simulink model "exp_one"  (R2017b)
settings: Solver=VariableStepAuto  StartTime=0.0  StopTime=0.1  RelTol=1e-3
libraries: powerlib x5, re_lib x1
settings Model: Creator=priya  LastModifiedBy=VIJAYPRASATH
settings DataIOCC: ReturnWorkspaceOutputs=on
settings DebuggingCC: UnconnectedInputMsg=none  UnconnectedOutputMsg=none  UnconnectedLineMsg=none
settings ModelReferenceCC: EnableRefExpFcnMdlSchedulingChecks=off
settings SFSimCC: SimUseLocalCustomCode=on
settings RTWCC: Description=Generic Real-Time Target  RTWUseLocalCustomCode=on

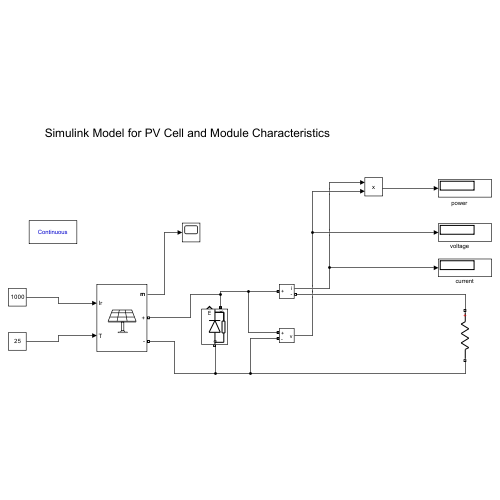
[thumbnail: Simulink's stored preview of the top-level diagram]
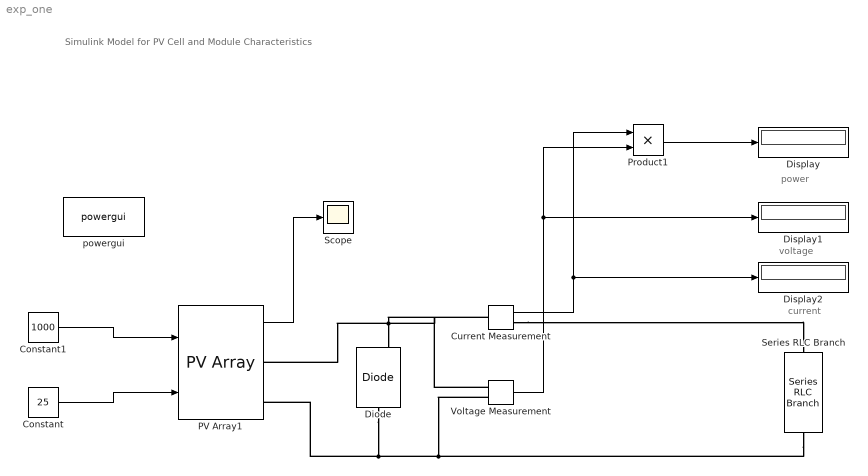
== system exp_one ==
  note: current
  note: voltage
  note: power
  note: Simulink Model for PV Cell and Module Characteristics
  Constant : Constant  Value=25
  Constant1 : Constant  Value=1000
  Current Measurement : powerlib/Measurements/Current Measurement  PhasorSimulation=off  OutputType=Complex  PSBequivalent=0
  Diode : powerlib/Power Electronics/Diode  Ron=0.001  Lon=0  Vf=0.7  IC=0  UseSnubber=0  Rs=500  Cs=250e-9  Measurements=on
  Display : Display
  Display1 : Display
  Display2 : Display
  PV Array1 : re_lib/Solar/PV Array  Npar=1  Nser=4  PlotType=array @ 1000 W/m2 & specified temperatures  S_vec="[ 1000  500  100 ]"  Temp_C_vec="[ 45 25  ]"  ModuleName=Trina Solar TSM-350DEG14(II)  PlotWhenSelected=off  Pm=349.965  Ncell=72  Voc=46.9  Isc=9.6  Vm=38.5  Im=9.09  beta_Voc_pc=-0.3014  alpha_Isc_pc=0.054604  beta_Voc=-0.14136  alpha_Isc=0.005242  IL=9.6084  I0=3.5075e-11  nI=0.96299  Rsh=597.8018  Rs=0.32702  RobustModel=off  RobustCellTemperature=313.3991  BAL=on  Tc=1e-6  Tfilter=5e-5
  Product1 : Product
  Scope : Scope
  Series RLC Branch : powerlib/Elements/Series RLC Branch  LConnTagsString=__new0  RConnTagsString=__new0  BranchType=R  Resistance=16  Inductance=1e-3  SetiL0=off  InitialCurrent=0  Capacitance=1e-6  Setx0=off  InitialVoltage=0  Measurements=None
  Voltage Measurement : powerlib/Measurements/Voltage Measurement  PhasorSimulation=off  OutputType=Complex  PSBequivalent=0
  powergui : powerlib/powergui  Priority=1  SimulationMode=Continuous  SampleTime=50e-6  frequency=60  Iterations=50  frequencyindice=0  Pbase=100e6  ErrMax=1e-4  UnitsV=kV  UnitsW=MW  buscounter=0  FunctionMessages=off  echomessages=off  EnableUseOfTLC=off  CurrentSourceSwitches=off  DisableSnubberDevices=off  DisableRonSwitches=off  DisableVfSwitches=off  DisplayEquations=off  AutomaticDiscreteSolvers=off  SolverType=Tustin/Backward Euler (TBE)  Interpol=off  ExternalGateDelay=off  methode=off  Ts=100  x0status=blocks  SPID=on  SwTol=0  HookPort=off  NonlinearTolerance=1e-4  nMaxIteration=100  ContinueOnMaxIteration=off  RestoreLinks=warning  ResistiveCurrentMeasurement=off  Frange=[0:2:500]  Ylog=off  Xlog=on  ShowGrid=off  save=off  variable=ZData  structure=0  ZoomFFT=off  StartTime=0.0  cycles=1  DisplayStyle=1  fundamental=60  FreqAxis=off  MaxFrequency=1000  frequencyindicesteady=1  RmsSteady=1  display=off
  wires:
  PV Array1/1 -> Scope/1
  Constant1/1 -> PV Array1/1
  Constant/1 -> PV Array1/2
  Current Measurement/1 -> Product1/1, Display2/1
  Voltage Measurement/1 -> Display1/1, Product1/2
  Product1/1 -> Display/1
  connections:
  Voltage Measurement/LConn1 -- Current Measurement/LConn1 -- PV Array1/RConn1 -- Diode/RConn1
  Current Measurement/RConn1 -- Series RLC Branch/LConn1
  Series RLC Branch/RConn1 -- Voltage Measurement/LConn2 -- PV Array1/RConn2 -- Diode/LConn1
